simulink model "A3_4_vrx"  (R2024b)
settings: Solver=ode4  StartTime=0.0  StopTime=T_run  FixedStep=Ts_ctrl  RelTol=1e-3
InitFcn:
  | if ~exist('A3_model_init','file'), addpath(fileparts(get_param('A3_4_vrx','FileName'))); end, A3_model_init('A3_4_vrx')
StopFcn:
  | A3_model_done('A3_4_vrx')
values from neighbouring files (symbols this model uses):
  alloc_mode = 2    [A3_setup.m]
  animate = 0    [A3_setup.m]
  az_prm = [half_beam; l_thr; F_max; d_max; rev_on]    [A3_setup.m]
  d_rate = deg2rad(d_rate_deg)    [A3_setup.m]
  F_max = 500    [A3_azpolar_example.m]    (also in A3_nullspace_example.m; A3_pinv_example.m; A3_setup.m)
  Kb = Ki_u/Kp_u    (= 0.333333333333)    [A3_setup.m]
  Kd_psi = 200    [A3_setup.m]
  Ki_u = 100    [A3_setup.m]
  Ki_v = 100    [A3_setup.m]
  Kp_psi = 400    [A3_setup.m]
  Kp_u = 300    [A3_setup.m]
  Kp_v = 300    [A3_setup.m]
  Kp_x = 0.4    [A3_setup.m]
  Kp_y = 0.4    [A3_setup.m]
  N_max = 2*half_beam*F_max    (= 1027.135)    [A3_setup.m]
  origin_east = 0    [A3_setup.m]
  origin_north = 0    [A3_setup.m]
  R_stop = 1.5    [A3_setup.m]
  stop_hold = 15    [A3_setup.m]
  stop_q = [x_d; y_d; psi_d]    [A3_setup.m]
  svo_rate = deg2rad(svo_rate_deg)    [A3_setup.m]
  svo_tau = svo_tau_s    (= 0.2)    [A3_setup.m]
  Ts_ctrl = 0.05    [A3_setup.m]
  u_max = 1.5    [A3_setup.m]
  U_stop = 0.05    [A3_setup.m]
  v_max = 0.6    [A3_setup.m]
  vrx_pos_sign = -1    [A3_setup.m]
  Y_max = F_max / T_per_Y    [A3_setup.m]
libraries: ros2lib x9, slpidlib x2
settings Model: Creator=admin  LastModifiedBy=admin

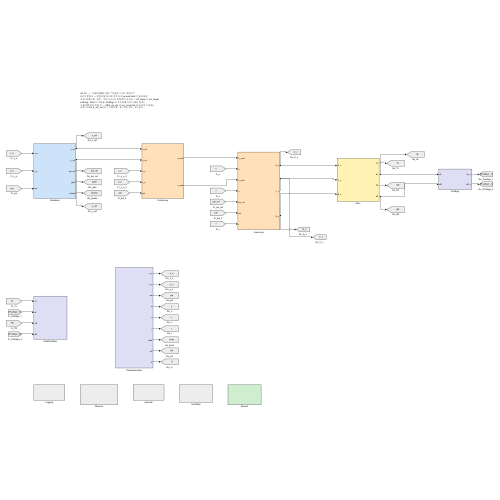
[thumbnail: Simulink's stored preview of the top-level diagram]
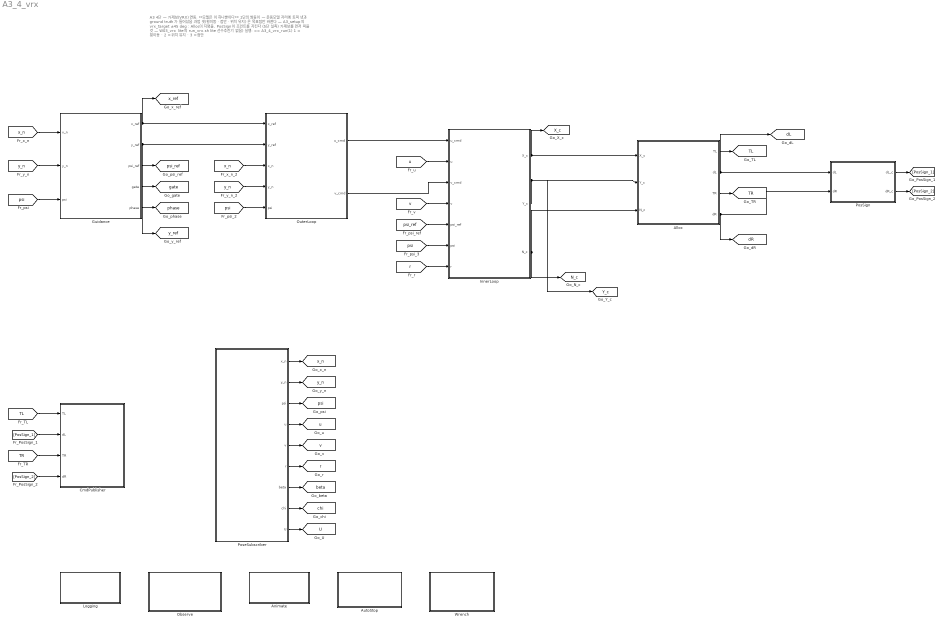
== system A3_4_vrx ==
  note: A3 4단  —  가제보(VRX) 연동. **모델은 이 하나뿐이다**
      | 2단의 쌍둥이 — 운동모델 자리에 토픽 넷과 ground truth 가 들어섰음
      | 과업 셋(횡이동 · 접안 · 위치 유지) 은 목표점만 바뀐다 — A3_setup 의 vrx_target
      | ±45 deg : Alloc 이 지령을, PosSign 이 조인트를 지킨다 (5단 실측)
      | 가제보를 먼저 띄울 것 — W03_vrx_lite 의 run_vrx.sh lite (선수추진기 없음)
      | 실행: >> A3_4_vrx_run(1)   1 = 횡이동 · 2 = 위치 유지 · 3 = 접안
  Alloc : Subsystem
  Animate : Subsystem
  AutoStop : Subsystem
  CmdPublisher : Subsystem
  Guidance : Subsystem
  InnerLoop : Subsystem
  Logging : Subsystem
  Observe : Subsystem
  OuterLoop : Subsystem
  PosSign : Subsystem
  PoseSubscriber : Subsystem
  Wrench : Subsystem
  tag scope: N_c=global, TL=global, TR=global, U=global, X_c=global, Y_c=global, beta=global, chi=global, dL=global, dR=global, gate=global, phase=global, psi=global, psi_ref=global, r=global, u=global, v=global, x_n=global, x_ref=global, y_n=global, y_ref=global
  wires:
  InnerLoop/2(Y_c) -> [Y_c], Alloc/2(Y_c)
  OuterLoop/1(u_cmd) -> InnerLoop/1(u_cmd)
  Alloc/2(dL) -> PosSign/1(dL), [dL]
  InnerLoop/1(X_c) -> Alloc/1(X_c), [X_c]
  OuterLoop/2(v_cmd) -> InnerLoop/3(v_cmd)
  Guidance/2(y_ref) -> OuterLoop/2(y_ref), [y_ref]
  Guidance/1(x_ref) -> OuterLoop/1(x_ref), [x_ref]
  PosSign/1(dL_c) -> [PosSign_1]
  PosSign/2(dR_c) -> [PosSign_2]
  Alloc/1(TL) -> [TL]
  Alloc/3(TR) -> [TR]
  PoseSubscriber/3(psi) -> [psi]
  Guidance/3(psi_ref) -> [psi_ref]
  PoseSubscriber/6(r) -> [r]
  PoseSubscriber/4(u) -> [u]
  PoseSubscriber/5(v) -> [v]
  PoseSubscriber/1(x_n) -> [x_n]
  PoseSubscriber/2(y_n) -> [y_n]
  [PosSign_1] -> CmdPublisher/2(dL)
  [PosSign_2] -> CmdPublisher/4(dR)
  [TL] -> CmdPublisher/1(TL)
  [TR] -> CmdPublisher/3(TR)
  [psi] -> Guidance/3(psi)
  [r] -> InnerLoop/7(r)
  [u] -> InnerLoop/2(u)
  [x_n] -> Guidance/1(x_n)
  [x_n] -> OuterLoop/3(x_n)
  [y_n] -> Guidance/2(y_n)
  [y_n] -> OuterLoop/4(y_n)
  PoseSubscriber/9(U) -> [U]
  PoseSubscriber/7(beta) -> [beta]
  PoseSubscriber/8(chi) -> [chi]
  Guidance/4(gate) -> [gate]
  Guidance/5(phase) -> [phase]
  [psi] -> OuterLoop/5(psi)
  [psi] -> InnerLoop/6(psi)
  [psi_ref] -> InnerLoop/5(psi_ref)
  [v] -> InnerLoop/4(v)
  Alloc/4(dR) -> [dR], PosSign/2(dR)
  InnerLoop/3(N_c) -> Alloc/3(N_c), [N_c]

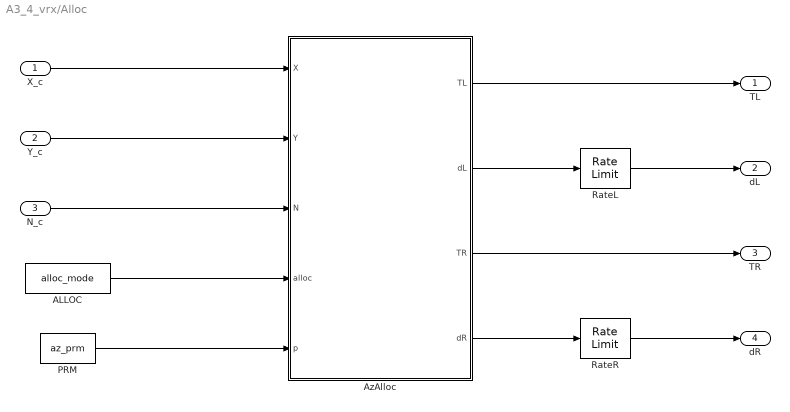
== system A3_4_vrx/Alloc ==
  X_c : Inport
  Y_c : Inport  Port=2
  N_c : Inport  Port=3
  ALLOC : Constant  Value=alloc_mode
  AzAlloc : MATLAB Function  TreatAsAtomicUnit=on
  PRM : Constant  Value=az_prm
  RateL : RateLimiter  RisingSlewLimit=d_rate  FallingSlewLimit=-d_rate  SampleTimeMode=inherited
  RateR : RateLimiter  RisingSlewLimit=d_rate  FallingSlewLimit=-d_rate  SampleTimeMode=inherited
  TL : Outport
  dL : Outport  Port=2
  TR : Outport  Port=3
  dR : Outport  Port=4
  wires:
  X_c/1 -> AzAlloc/1(X)
  Y_c/1 -> AzAlloc/2(Y)
  N_c/1 -> AzAlloc/3(N)
  ALLOC/1 -> AzAlloc/4(alloc)
  PRM/1 -> AzAlloc/5(p)
  AzAlloc/2(dL) -> RateL/1
  AzAlloc/4(dR) -> RateR/1
  AzAlloc/1(TL) -> TL/1
  RateL/1 -> dL/1
  RateR/1 -> dR/1
  AzAlloc/3(TR) -> TR/1

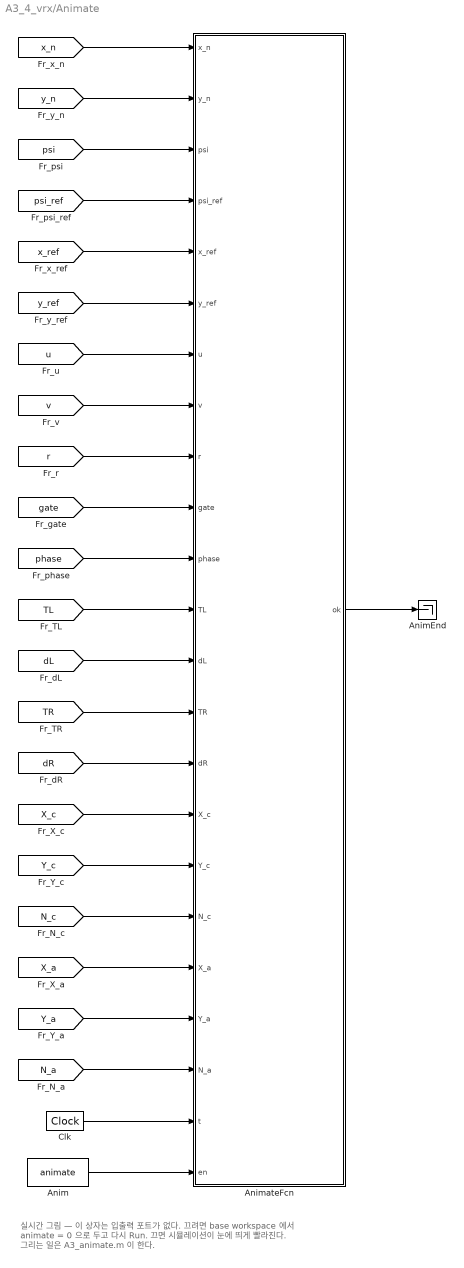
== system A3_4_vrx/Animate ==
  note: 실시간 그림 — 이 상자는 입출력 포트가 없다.
      | 끄려면 base workspace 에서  animate = 0  으로 두고 다시 Run.
      | 끄면 시뮬레이션이 눈에 띄게 빨라진다.
      | 그리는 일은 A3_animate.m 이 한다.
  Anim : Constant  Value=animate
  AnimEnd : Terminator
  AnimateFcn : MATLAB Function  TreatAsAtomicUnit=on
  Clk : DigitalClock  SampleTime=Ts_ctrl
  wires:
  [x_n] -> AnimateFcn/1(x_n)
  [y_n] -> AnimateFcn/2(y_n)
  [psi] -> AnimateFcn/3(psi)
  [psi_ref] -> AnimateFcn/4(psi_ref)
  [x_ref] -> AnimateFcn/5(x_ref)
  [y_ref] -> AnimateFcn/6(y_ref)
  [u] -> AnimateFcn/7(u)
  [v] -> AnimateFcn/8(v)
  [r] -> AnimateFcn/9(r)
  [gate] -> AnimateFcn/10(gate)
  [phase] -> AnimateFcn/11(phase)
  [TL] -> AnimateFcn/12(TL)
  [dL] -> AnimateFcn/13(dL)
  [TR] -> AnimateFcn/14(TR)
  [dR] -> AnimateFcn/15(dR)
  [X_c] -> AnimateFcn/16(X_c)
  [Y_c] -> AnimateFcn/17(Y_c)
  [N_c] -> AnimateFcn/18(N_c)
  [X_a] -> AnimateFcn/19(X_a)
  [Y_a] -> AnimateFcn/20(Y_a)
  [N_a] -> AnimateFcn/21(N_a)
  Clk/1 -> AnimateFcn/22(t)
  Anim/1 -> AnimateFcn/23(en)
  AnimateFcn/1(ok) -> AnimEnd/1

== system A3_4_vrx/AutoStop ==
  Done : RelationalOperator  OutDataTypeStr=boolean  RndMeth=Simplest  InputSameDT=off
  HeldFor : Integrator  ExternalReset=level
  Hold : Constant  Value=stop_hold
  One : Constant
  StopSim : Stop
  wires:
  One/1 -> HeldFor/1
  [gate] -> HeldFor/2
  HeldFor/1 -> Done/1
  Hold/1 -> Done/2
  Done/1 -> StopSim/1

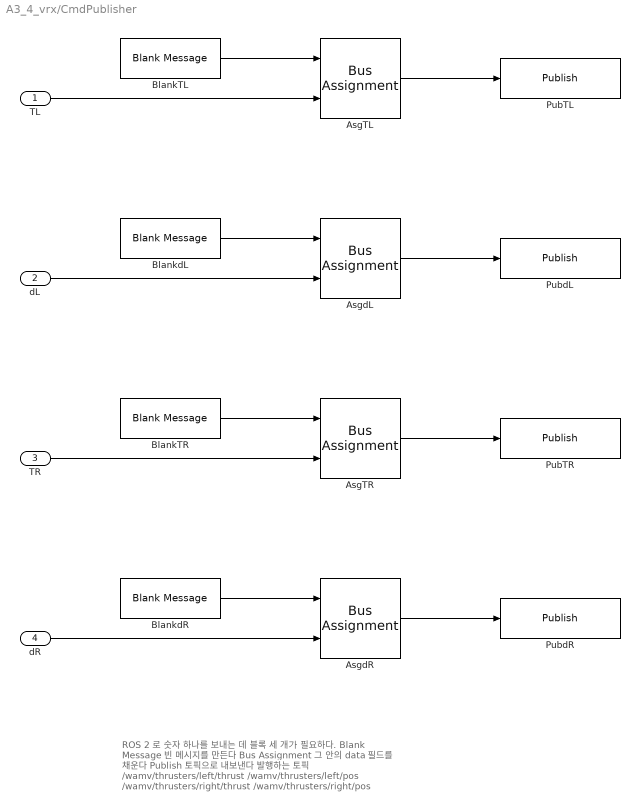
== system A3_4_vrx/CmdPublisher ==
  note: ROS 2 로 숫자 하나를 보내는 데 블록 세 개가 필요하다.
      |   Blank Message   빈 메시지를 만든다
      |   Bus Assignment  그 안의 data 필드를 채운다
      |   Publish         토픽으로 내보낸다
      |
      | 발행하는 토픽
      | /wamv/thrusters/left/thrust
      | /wamv/thrusters/left/pos
      | /wamv/thrusters/right/thrust
      | /wamv/thrusters/right/pos
  TL : Inport
  dL : Inport  Port=2
  TR : Inport  Port=3
  dR : Inport  Port=4
  AsgTL : BusAssignment  AssignedSignals=data
  AsgTR : BusAssignment  AssignedSignals=data
  AsgdL : BusAssignment  AssignedSignals=data
  AsgdR : BusAssignment  AssignedSignals=data
  BlankTL : ros2lib/Blank Message  messageClass=Message  entityType=std_msgs/Float64  messageType=std_msgs/Float64  SampleTime=Ts_ctrl
  BlankTR : ros2lib/Blank Message  messageClass=Message  entityType=std_msgs/Float64  messageType=std_msgs/Float64  SampleTime=Ts_ctrl
  BlankdL : ros2lib/Blank Message  messageClass=Message  entityType=std_msgs/Float64  messageType=std_msgs/Float64  SampleTime=Ts_ctrl
  BlankdR : ros2lib/Blank Message  messageClass=Message  entityType=std_msgs/Float64  messageType=std_msgs/Float64  SampleTime=Ts_ctrl
  PubTL : ros2lib/Publish  topicSource=Specify your own  topic=/wamv/thrusters/left/thrust  messageType=std_msgs/Float64  QOSHistory=Keep last  QOSDepth=1  QOSReliability=Reliable  QOSDurability=Volatile  QOSDeadline=Inf  QOSLifespan=Inf  QOSLiveliness=Automatic  QOSLeaseDuration=Inf  QOSAvoidROSNamespaceConventions=off
  PubTR : ros2lib/Publish  topicSource=Specify your own  topic=/wamv/thrusters/right/thrust  messageType=std_msgs/Float64  QOSHistory=Keep last  QOSDepth=1  QOSReliability=Reliable  QOSDurability=Volatile  QOSDeadline=Inf  QOSLifespan=Inf  QOSLiveliness=Automatic  QOSLeaseDuration=Inf  QOSAvoidROSNamespaceConventions=off
  PubdL : ros2lib/Publish  topicSource=Specify your own  topic=/wamv/thrusters/left/pos  messageType=std_msgs/Float64  QOSHistory=Keep last  QOSDepth=1  QOSReliability=Reliable  QOSDurability=Volatile  QOSDeadline=Inf  QOSLifespan=Inf  QOSLiveliness=Automatic  QOSLeaseDuration=Inf  QOSAvoidROSNamespaceConventions=off
  PubdR : ros2lib/Publish  topicSource=Specify your own  topic=/wamv/thrusters/right/pos  messageType=std_msgs/Float64  QOSHistory=Keep last  QOSDepth=1  QOSReliability=Reliable  QOSDurability=Volatile  QOSDeadline=Inf  QOSLifespan=Inf  QOSLiveliness=Automatic  QOSLeaseDuration=Inf  QOSAvoidROSNamespaceConventions=off
  wires:
  BlankTL/1 -> AsgTL/1
  AsgTL/1 -> PubTL/1
  TL/1 -> AsgTL/2
  BlankdL/1 -> AsgdL/1
  AsgdL/1 -> PubdL/1
  dL/1 -> AsgdL/2
  BlankTR/1 -> AsgTR/1
  AsgTR/1 -> PubTR/1
  TR/1 -> AsgTR/2
  BlankdR/1 -> AsgdR/1
  AsgdR/1 -> PubdR/1
  dR/1 -> AsgdR/2

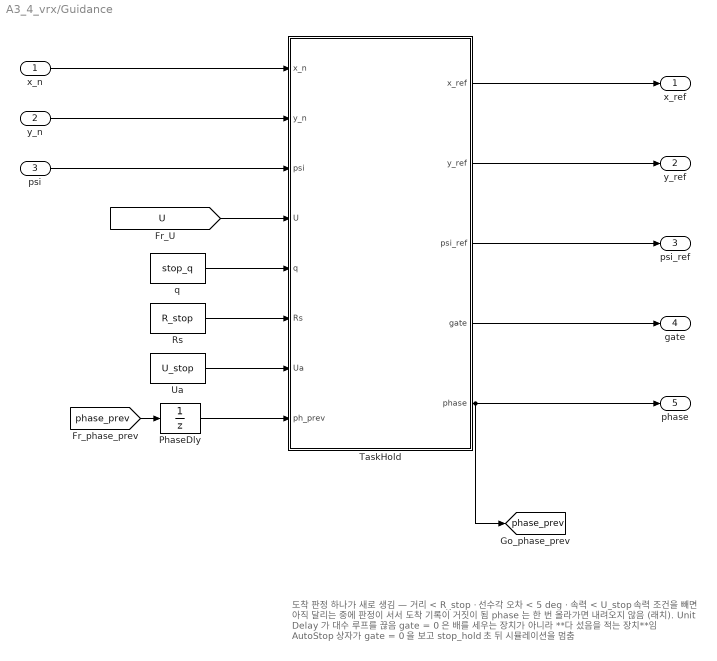
== system A3_4_vrx/Guidance ==
  note: 도착 판정 하나가 새로 생김 — 거리 < R_stop · 선수각 오차 < 5 deg · 속력 < U_stop
      | 속력 조건을 빼면 아직 달리는 중에 판정이 서서 도착 기록이 거짓이 됨
      | phase 는 한 번 올라가면 내려오지 않음 (래치). Unit Delay 가 대수 루프를 끊음
      | gate = 0 은 배를 세우는 장치가 아니라 **다 섰음을 적는 장치**임
      | AutoStop 상자가 gate = 0 을 보고 stop_hold 초 뒤 시뮬레이션을 멈춤
  x_n : Inport
  y_n : Inport  Port=2
  psi : Inport  Port=3
  PhaseDly : UnitDelay  Description=phase 래치가 자기 자신을 입력으로 받으므로 그대로 되먹이면 대수 루프가 된다. 한 스텝 전 값을 쓰는 것 말고는 끊을 방법이 없는 자리다. 표본 간격을 고정 스텝(Ts_ctrl)과 같게 두어 연속 솔버(ode4)와 어긋나지 않는다.  SampleTime=Ts_ctrl  HasFrameUpgradeWarning=on
  Rs : Constant  Value=R_stop
  TaskHold : MATLAB Function  TreatAsAtomicUnit=on
  Ua : Constant  Value=U_stop
  q : Constant  Value=stop_q
  x_ref : Outport
  y_ref : Outport  Port=2
  psi_ref : Outport  Port=3
  gate : Outport  Port=4
  phase : Outport  Port=5
  tag scope: phase_prev=global
  wires:
  x_n/1 -> TaskHold/1(x_n)
  y_n/1 -> TaskHold/2(y_n)
  psi/1 -> TaskHold/3(psi)
  [U] -> TaskHold/4(U)
  q/1 -> TaskHold/5(q)
  Rs/1 -> TaskHold/6(Rs)
  Ua/1 -> TaskHold/7(Ua)
  PhaseDly/1 -> TaskHold/8(ph_prev)
  TaskHold/1(x_ref) -> x_ref/1
  TaskHold/2(y_ref) -> y_ref/1
  TaskHold/3(psi_ref) -> psi_ref/1
  TaskHold/4(gate) -> gate/1
  TaskHold/5(phase) -> phase/1, [phase_prev]
  [phase_prev] -> PhaseDly/1

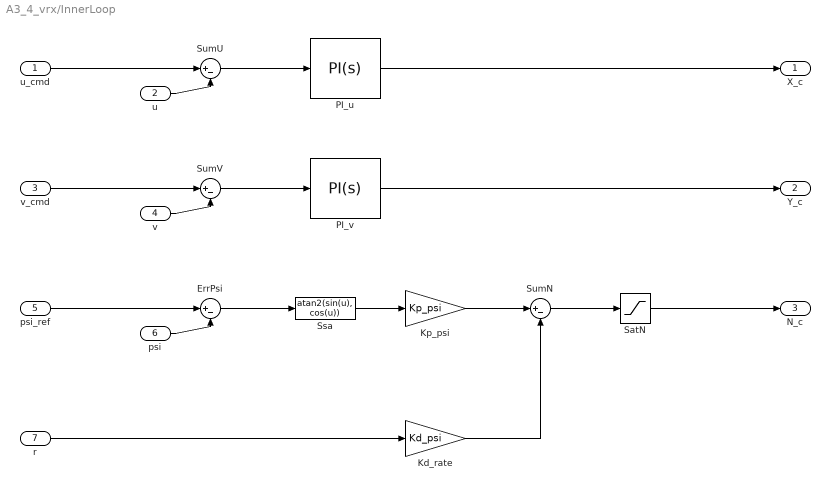
== system A3_4_vrx/InnerLoop ==
  u_cmd : Inport
  u : Inport  Port=2
  v_cmd : Inport  Port=3
  v : Inport  Port=4
  psi_ref : Inport  Port=5
  psi : Inport  Port=6
  r : Inport  Port=7
  ErrPsi : Sum  Inputs=|+-
  Kd_rate : Gain  Gain=Kd_psi
  Kp_psi : Gain  Gain=Kp_psi
  PI_u : slpidlib/PID Controller  Controller=PI  Form=Parallel  TimeDomain=Continuous-time  UseExternalTs=off  SampleTime=-1  IntegratorMethod=Forward Euler  FilterMethod=Forward Euler  ControllerParametersSource=internal  P=Kp_u  I=Ki_u  UseKiTs=off  D=0  UseExternalDerivativeSource=off  N=100  UseFilter=on  TunerSelectOption=Transfer Function Based (PID Tuner App)  InitialConditionSource=internal  InitialConditionForIntegrator=0  InitialConditionForFilter=0  DifferentiatorICPrevScaledInput=0  ExternalReset=none  TrackingMode=off  Kt=1  LimitOutput=on  SatLimitsSource=internal  UpperSaturationLimit=2*F_max  LowerSaturationLimit=-(2*F_max)  LinearizeAsGain=on  AntiWindupMode=back-calculation  Kb=Kb  LimitIntegrator=off  UpperIntegratorSaturationLimit=inf  LowerIntegratorSaturationLimit=-inf  POutMin=[]  POutMax=[]  IOutMin=[]  IOutMax=[]  DOutMin=[]  DOutMax=[]  NOutMin=[]  NOutMax=[]  SumOutMin=[]  SumOutMax=[]  SaturationOutMin=[]  SaturationOutMax=[]  PParamMin=[]  PParamMax=[]  IParamMin=[]  IParamMax=[]  DParamMin=[]  DParamMax=[]  NParamMin=[]  NParamMax=[]  KbParamMin=[]  KbParamMax=[]  KtParamMin=[]  KtParamMax=[]  KbOutMin=[]  KbOutMax=[]  KtOutMin=[]  KtOutMax=[]  IntegratorOutMin=[]  IntegratorOutMax=[]  FilterOutMin=[]  FilterOutMax=[]  SumI1OutMin=[]  SumI1OutMax=[]  SumI2OutMin=[]  SumI2OutMax=[]  SumI3OutMin=[]  SumI3OutMax=[]  SumI4OutMin=[]  SumI4OutMax=[]  SumDOutMin=[]  SumDOutMax=[]  DifferentiatorOutMin=[]  DifferentiatorOutMax=[]  FilterDiffOutCoefMin=[]  FilterDiffOutCoefMax=[]  ReciprocalOutMin=[]  ReciprocalOutMax=[]  SumDenOutMin=[]  SumDenOutMax=[]  SumNumOutMin=[]  SumNumOutMax=[]  DivideOutMin=[]  DivideOutMax=[]  UdiffTsProdOutMin=[]  UdiffTsProdOutMax=[]  NTsProdOutMin=[]  NTsProdOutMax=[]  UintegralTsProdOutMin=[]  UintegralTsProdOutMax=[]  UngainTsProdOutMin=[]  UngainTsProdOutMax=[]  ClampingZeroOutDataTypeStr=Inherit: Inherit via back propagation  ClampingZeroOutMin=[]  ClampingZeroOutMax=[]  FilterDenConstantOutDataTypeStr=Inherit: Inherit via back propagation  FilterDenConstantOutMin=[]  FilterDenConstantOutMax=[]  PCopyOutDataTypeStr=Inherit: Inherit via back propagation  PCopyOutMin=[]  PCopyOutMax=[]  NCopyOutDataTypeStr=Inherit: Inherit via back propagation  NCopyOutMin=[]  NCopyOutMax=[]  IntegratorContinuousStateAttributes=''  IntegratorStateMustResolveToSignalObject=off  IntegratorRTWStateStorageClass=Auto  FilterContinuousStateAttributes=''  FilterStateMustResolveToSignalObject=off  FilterRTWStateStorageClass=Auto  ParallelPVariant=InternalParameters  IdealPVariant=Disabled  IVariant=InternalParameters  DVariant=Disabled  IntegratorVariant=Continuous  SatVariant=Enabled  AWVariant=BackCalculation  PCopyVariant=Disabled  TRVariant=Disabled  FdbkBlocksVariant=Forward  IdealPFdbkVariant=Disabled  SatFdbkVariant=Disabled  DerivativeFilterVariant=Disabled  NVariant=Disabled  NCopyVariant=Disabled_SignalSpec  FilterICVariant=Disabled  IntegratorICVariant=InternalICs  ExternalResetVariant=Disabled  TRSumVariant=Passthrough  SumFdbkVariant=Disabled  SumVariant=Sum_PI  TsampFilterVariant=InternalTs  TsampNgainVariant=Passthrough  TsampIntegralVariant=Disabled_SignalSpec  ExternalSaturationOutDataTypeStr=Inherit: Same as second input  DerivativeSourceVariant=Disabled  PreIntVariant=InternalPreInt
  PI_v : slpidlib/PID Controller  Controller=PI  Form=Parallel  TimeDomain=Continuous-time  UseExternalTs=off  SampleTime=-1  IntegratorMethod=Forward Euler  FilterMethod=Forward Euler  ControllerParametersSource=internal  P=Kp_v  I=Ki_v  UseKiTs=off  D=0  UseExternalDerivativeSource=off  N=100  UseFilter=on  TunerSelectOption=Transfer Function Based (PID Tuner App)  InitialConditionSource=internal  InitialConditionForIntegrator=0  InitialConditionForFilter=0  DifferentiatorICPrevScaledInput=0  ExternalReset=none  TrackingMode=off  Kt=1  LimitOutput=on  SatLimitsSource=internal  UpperSaturationLimit=Y_max  LowerSaturationLimit=-(Y_max)  LinearizeAsGain=on  AntiWindupMode=back-calculation  Kb=Kb  LimitIntegrator=off  UpperIntegratorSaturationLimit=inf  LowerIntegratorSaturationLimit=-inf  POutMin=[]  POutMax=[]  IOutMin=[]  IOutMax=[]  DOutMin=[]  DOutMax=[]  NOutMin=[]  NOutMax=[]  SumOutMin=[]  SumOutMax=[]  SaturationOutMin=[]  SaturationOutMax=[]  PParamMin=[]  PParamMax=[]  IParamMin=[]  IParamMax=[]  DParamMin=[]  DParamMax=[]  NParamMin=[]  NParamMax=[]  KbParamMin=[]  KbParamMax=[]  KtParamMin=[]  KtParamMax=[]  KbOutMin=[]  KbOutMax=[]  KtOutMin=[]  KtOutMax=[]  IntegratorOutMin=[]  IntegratorOutMax=[]  FilterOutMin=[]  FilterOutMax=[]  SumI1OutMin=[]  SumI1OutMax=[]  SumI2OutMin=[]  SumI2OutMax=[]  SumI3OutMin=[]  SumI3OutMax=[]  SumI4OutMin=[]  SumI4OutMax=[]  SumDOutMin=[]  SumDOutMax=[]  DifferentiatorOutMin=[]  DifferentiatorOutMax=[]  FilterDiffOutCoefMin=[]  FilterDiffOutCoefMax=[]  ReciprocalOutMin=[]  ReciprocalOutMax=[]  SumDenOutMin=[]  SumDenOutMax=[]  SumNumOutMin=[]  SumNumOutMax=[]  DivideOutMin=[]  DivideOutMax=[]  UdiffTsProdOutMin=[]  UdiffTsProdOutMax=[]  NTsProdOutMin=[]  NTsProdOutMax=[]  UintegralTsProdOutMin=[]  UintegralTsProdOutMax=[]  UngainTsProdOutMin=[]  UngainTsProdOutMax=[]  ClampingZeroOutDataTypeStr=Inherit: Inherit via back propagation  ClampingZeroOutMin=[]  ClampingZeroOutMax=[]  FilterDenConstantOutDataTypeStr=Inherit: Inherit via back propagation  FilterDenConstantOutMin=[]  FilterDenConstantOutMax=[]  PCopyOutDataTypeStr=Inherit: Inherit via back propagation  PCopyOutMin=[]  PCopyOutMax=[]  NCopyOutDataTypeStr=Inherit: Inherit via back propagation  NCopyOutMin=[]  NCopyOutMax=[]  IntegratorContinuousStateAttributes=''  IntegratorStateMustResolveToSignalObject=off  IntegratorRTWStateStorageClass=Auto  FilterContinuousStateAttributes=''  FilterStateMustResolveToSignalObject=off  FilterRTWStateStorageClass=Auto  ParallelPVariant=InternalParameters  IdealPVariant=Disabled  IVariant=InternalParameters  DVariant=Disabled  IntegratorVariant=Continuous  SatVariant=Enabled  AWVariant=BackCalculation  PCopyVariant=Disabled  TRVariant=Disabled  FdbkBlocksVariant=Forward  IdealPFdbkVariant=Disabled  SatFdbkVariant=Disabled  DerivativeFilterVariant=Disabled  NVariant=Disabled  NCopyVariant=Disabled_SignalSpec  FilterICVariant=Disabled  IntegratorICVariant=InternalICs  ExternalResetVariant=Disabled  TRSumVariant=Passthrough  SumFdbkVariant=Disabled  SumVariant=Sum_PI  TsampFilterVariant=InternalTs  TsampNgainVariant=Passthrough  TsampIntegralVariant=Disabled_SignalSpec  ExternalSaturationOutDataTypeStr=Inherit: Same as second input  DerivativeSourceVariant=Disabled  PreIntVariant=InternalPreInt
  SatN : Saturate  UpperLimit=N_max  LowerLimit=-(N_max)
  Ssa : Fcn  Expr=atan2(sin(u), cos(u))
  SumN : Sum  Inputs=|+-
  SumU : Sum  Inputs=|+-
  SumV : Sum  Inputs=|+-
  X_c : Outport
  Y_c : Outport  Port=2
  N_c : Outport  Port=3
  wires:
  u_cmd/1 -> SumU/1
  u/1 -> SumU/2
  v_cmd/1 -> SumV/1
  v/1 -> SumV/2
  SumU/1 -> PI_u/1
  SumV/1 -> PI_v/1
  ErrPsi/1 -> Ssa/1
  psi_ref/1 -> ErrPsi/1
  psi/1 -> ErrPsi/2
  Ssa/1 -> Kp_psi/1
  r/1 -> Kd_rate/1
  Kp_psi/1 -> SumN/1
  Kd_rate/1 -> SumN/2
  SumN/1 -> SatN/1
  PI_u/1 -> X_c/1
  SatN/1 -> N_c/1
  PI_v/1 -> Y_c/1

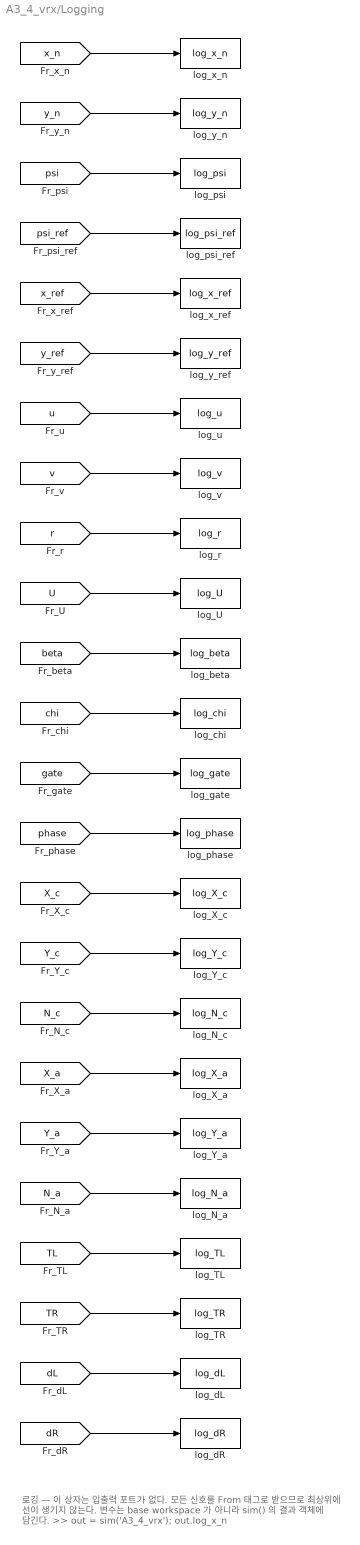
== system A3_4_vrx/Logging ==
  note: 로깅 — 이 상자는 입출력 포트가 없다.
      | 모든 신호를 From 태그로 받으므로 최상위에 선이 생기지 않는다.
      | 변수는 base workspace 가 아니라 sim() 의 결과 객체에 담긴다.
      |   >> out = sim('A3_4_vrx');  out.log_x_n
  log_N_a : ToWorkspace  VariableName=log_N_a  SaveFormat=Timeseries  SampleTime=Ts_ctrl
  log_N_c : ToWorkspace  VariableName=log_N_c  SaveFormat=Timeseries  SampleTime=Ts_ctrl
  log_TL : ToWorkspace  VariableName=log_TL  SaveFormat=Timeseries  SampleTime=Ts_ctrl
  log_TR : ToWorkspace  VariableName=log_TR  SaveFormat=Timeseries  SampleTime=Ts_ctrl
  log_U : ToWorkspace  VariableName=log_U  SaveFormat=Timeseries  SampleTime=Ts_ctrl
  log_X_a : ToWorkspace  VariableName=log_X_a  SaveFormat=Timeseries  SampleTime=Ts_ctrl
  log_X_c : ToWorkspace  VariableName=log_X_c  SaveFormat=Timeseries  SampleTime=Ts_ctrl
  log_Y_a : ToWorkspace  VariableName=log_Y_a  SaveFormat=Timeseries  SampleTime=Ts_ctrl
  log_Y_c : ToWorkspace  VariableName=log_Y_c  SaveFormat=Timeseries  SampleTime=Ts_ctrl
  log_beta : ToWorkspace  VariableName=log_beta  SaveFormat=Timeseries  SampleTime=Ts_ctrl
  log_chi : ToWorkspace  VariableName=log_chi  SaveFormat=Timeseries  SampleTime=Ts_ctrl
  log_dL : ToWorkspace  VariableName=log_dL  SaveFormat=Timeseries  SampleTime=Ts_ctrl
  log_dR : ToWorkspace  VariableName=log_dR  SaveFormat=Timeseries  SampleTime=Ts_ctrl
  log_gate : ToWorkspace  VariableName=log_gate  SaveFormat=Timeseries  SampleTime=Ts_ctrl
  log_phase : ToWorkspace  VariableName=log_phase  SaveFormat=Timeseries  SampleTime=Ts_ctrl
  log_psi : ToWorkspace  VariableName=log_psi  SaveFormat=Timeseries  SampleTime=Ts_ctrl
  log_psi_ref : ToWorkspace  VariableName=log_psi_ref  SaveFormat=Timeseries  SampleTime=Ts_ctrl
  log_r : ToWorkspace  VariableName=log_r  SaveFormat=Timeseries  SampleTime=Ts_ctrl
  log_u : ToWorkspace  VariableName=log_u  SaveFormat=Timeseries  SampleTime=Ts_ctrl
  log_v : ToWorkspace  VariableName=log_v  SaveFormat=Timeseries  SampleTime=Ts_ctrl
  log_x_n : ToWorkspace  VariableName=log_x_n  SaveFormat=Timeseries  SampleTime=Ts_ctrl
  log_x_ref : ToWorkspace  VariableName=log_x_ref  SaveFormat=Timeseries  SampleTime=Ts_ctrl
  log_y_n : ToWorkspace  VariableName=log_y_n  SaveFormat=Timeseries  SampleTime=Ts_ctrl
  log_y_ref : ToWorkspace  VariableName=log_y_ref  SaveFormat=Timeseries  SampleTime=Ts_ctrl
  wires:
  [x_n] -> log_x_n/1
  [y_n] -> log_y_n/1
  [psi] -> log_psi/1
  [psi_ref] -> log_psi_ref/1
  [x_ref] -> log_x_ref/1
  [y_ref] -> log_y_ref/1
  [u] -> log_u/1
  [v] -> log_v/1
  [r] -> log_r/1
  [U] -> log_U/1
  [beta] -> log_beta/1
  [chi] -> log_chi/1
  [gate] -> log_gate/1
  [phase] -> log_phase/1
  [X_c] -> log_X_c/1
  [Y_c] -> log_Y_c/1
  [N_c] -> log_N_c/1
  [X_a] -> log_X_a/1
  [Y_a] -> log_Y_a/1
  [N_a] -> log_N_a/1
  [TL] -> log_TL/1
  [TR] -> log_TR/1
  [dL] -> log_dL/1
  [dR] -> log_dR/1

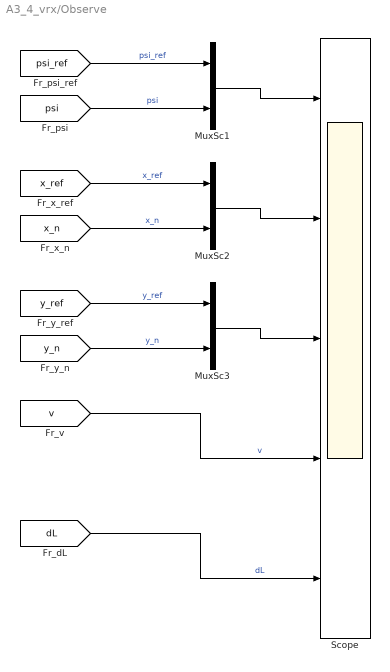
== system A3_4_vrx/Observe ==
  MuxSc1 : Mux  Inputs=2
  MuxSc2 : Mux  Inputs=2
  MuxSc3 : Mux  Inputs=2
  Scope : Scope  NumInputPorts=5
  wires:
  [psi_ref] -> MuxSc1/1  "psi_ref"
  [psi] -> MuxSc1/2  "psi"
  MuxSc1/1 -> Scope/1
  [x_ref] -> MuxSc2/1  "x_ref"
  [x_n] -> MuxSc2/2  "x_n"
  MuxSc2/1 -> Scope/2
  [y_ref] -> MuxSc3/1  "y_ref"
  [y_n] -> MuxSc3/2  "y_n"
  MuxSc3/1 -> Scope/3
  [v] -> Scope/4  "v"
  [dL] -> Scope/5  "dL"

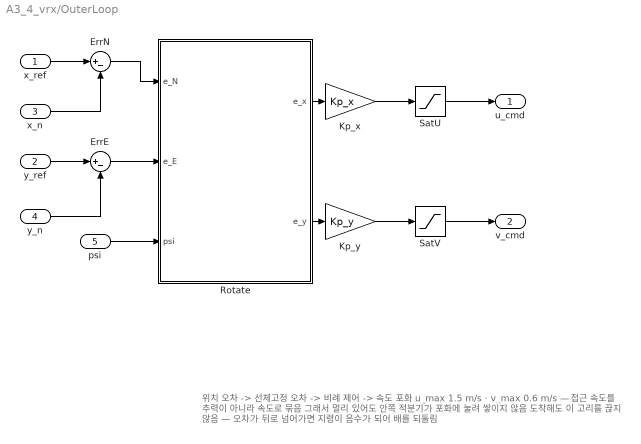
== system A3_4_vrx/OuterLoop ==
  note: 위치 오차 -> 선체고정 오차 -> 비례 제어 -> 속도 포화
      | u_max 1.5 m/s · v_max 0.6 m/s — 접근 속도를 추력이 아니라 속도로 묶음
      | 그래서 멀리 있어도 안쪽 적분기가 포화에 눌려 쌓이지 않음
      | 도착해도 이 고리를 끊지 않음 — 오차가 뒤로 넘어가면 지령이 음수가 되어 배를 되돌림
  x_ref : Inport
  y_ref : Inport  Port=2
  x_n : Inport  Port=3
  y_n : Inport  Port=4
  psi : Inport  Port=5
  ErrE : Sum  Inputs=|+-
  ErrN : Sum  Inputs=|+-
  Kp_x : Gain  Gain=Kp_x
  Kp_y : Gain  Gain=Kp_y
  Rotate : MATLAB Function  TreatAsAtomicUnit=on
  SatU : Saturate  UpperLimit=u_max  LowerLimit=-(u_max)
  SatV : Saturate  UpperLimit=v_max  LowerLimit=-(v_max)
  u_cmd : Outport
  v_cmd : Outport  Port=2
  wires:
  x_ref/1 -> ErrN/1
  x_n/1 -> ErrN/2
  ErrE/1 -> Rotate/2(e_E)
  y_ref/1 -> ErrE/1
  y_n/1 -> ErrE/2
  Rotate/1(e_x) -> Kp_x/1
  ErrN/1 -> Rotate/1(e_N)
  psi/1 -> Rotate/3(psi)
  Rotate/2(e_y) -> Kp_y/1
  Kp_x/1 -> SatU/1
  Kp_y/1 -> SatV/1
  SatU/1 -> u_cmd/1
  SatV/1 -> v_cmd/1

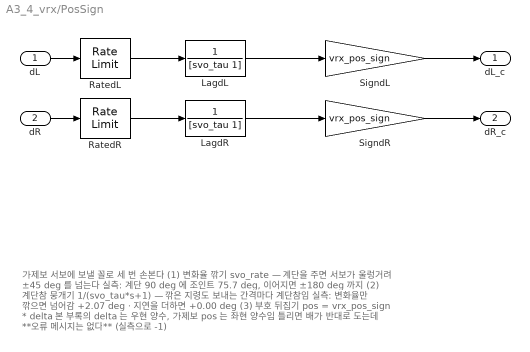
== system A3_4_vrx/PosSign ==
  note: 가제보 서보에 보낼 꼴로 세 번 손본다
      | (1) 변화율 깎기 svo_rate — 계단을 주면 서보가 울렁거려 ±45 deg 를 넘는다
      |       실측: 계단 90 deg 에 조인트 75.7 deg, 이어지면 ±180 deg 까지
      | (2) 계단참 뭉개기 1/(svo_tau*s+1) — 깎은 지령도 보내는 간격마다 계단참임
      |       실측: 변화율만 깎으면 넘어감 +2.07 deg · 지연을 더하면 +0.00 deg
      | (3) 부호 뒤집기 pos = vrx_pos_sign * delta
      |       본 부록의 delta 는 우현 양수, 가제보 pos 는 좌현 양수임
      |       틀리면 배가 반대로 도는데 **오류 메시지는 없다** (실측으로 -1)
  dL : Inport
  dR : Inport  Port=2
  LagdL : TransferFcn  Denominator=[svo_tau 1]
  LagdR : TransferFcn  Denominator=[svo_tau 1]
  RatedL : RateLimiter  RisingSlewLimit=svo_rate  FallingSlewLimit=-svo_rate  SampleTimeMode=inherited
  RatedR : RateLimiter  RisingSlewLimit=svo_rate  FallingSlewLimit=-svo_rate  SampleTimeMode=inherited
  SigndL : Gain  Gain=vrx_pos_sign
  SigndR : Gain  Gain=vrx_pos_sign
  dL_c : Outport
  dR_c : Outport  Port=2
  wires:
  dL/1 -> RatedL/1
  RatedL/1 -> LagdL/1
  LagdL/1 -> SigndL/1
  SigndL/1 -> dL_c/1
  dR/1 -> RatedR/1
  RatedR/1 -> LagdR/1
  LagdR/1 -> SigndR/1
  SigndR/1 -> dR_c/1

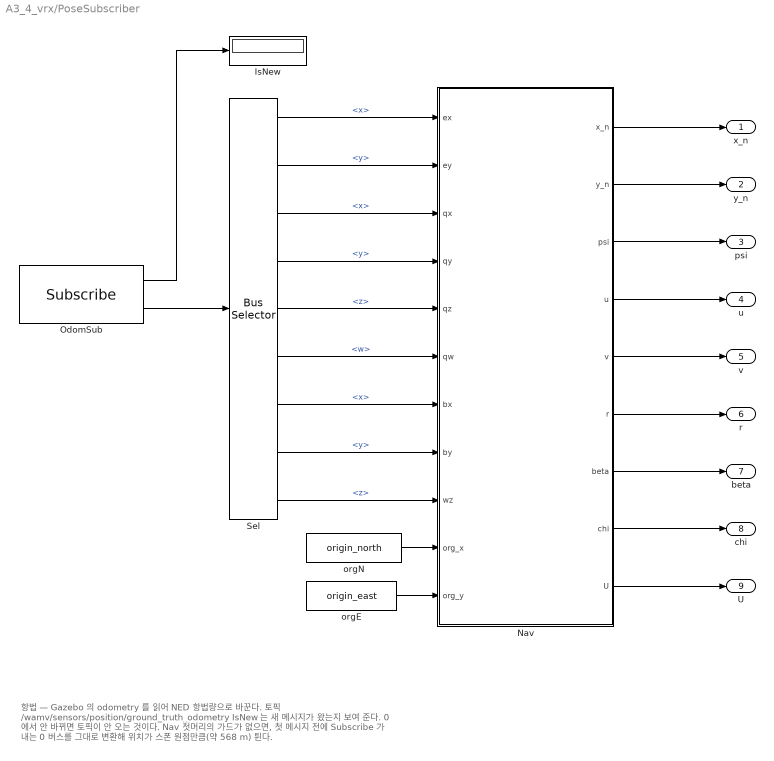
== system A3_4_vrx/PoseSubscriber ==
  note: 항법 — Gazebo 의 odometry 를 읽어 NED 항법량으로 바꾼다.
      |   토픽 /wamv/sensors/position/ground_truth_odometry
      |
      | IsNew 는 새 메시지가 왔는지 보여 준다. 0 에서 안 바뀌면 토픽이 안 오는 것이다.
      | Nav 첫머리의 가드가 없으면, 첫 메시지 전에 Subscribe 가 내는 0 버스를
      | 그대로 변환해 위치가 스폰 원점만큼(약 568 m) 튄다.
  IsNew : Display
  Nav : MATLAB Function  TreatAsAtomicUnit=on
  OdomSub : ros2lib/Subscribe  topicSource=Specify your own  topic=/wamv/sensors/position/ground_truth_odometry  messageType=nav_msgs/Odometry  sampleTime=Ts_ctrl  QOSHistory=Keep last  QOSDepth=1  QOSReliability=Reliable  QOSDurability=Volatile  QOSDeadline=Inf  QOSLifespan=Inf  QOSLiveliness=Automatic  QOSLeaseDuration=Inf  QOSAvoidROSNamespaceConventions=off
  Sel : BusSelector  OutputSignals=pose.pose.position.x,pose.pose.position.y,pose.pose.orientation.x,pose.pose.orientation.y,pose.pose.orientation.z,pose.pose.orientation.w,twist.twist.linear.x,twist.twist.linear.y,twist.twist.angular.z
  orgE : Constant  Value=origin_east
  orgN : Constant  Value=origin_north
  x_n : Outport
  y_n : Outport  Port=2
  psi : Outport  Port=3
  u : Outport  Port=4
  v : Outport  Port=5
  r : Outport  Port=6
  beta : Outport  Port=7
  chi : Outport  Port=8
  U : Outport  Port=9
  wires:
  OdomSub/1 -> IsNew/1
  OdomSub/2 -> Sel/1
  Sel/1 -> Nav/1(ex)  "<x>"
  Sel/2 -> Nav/2(ey)  "<y>"
  Sel/3 -> Nav/3(qx)  "<x>"
  Sel/4 -> Nav/4(qy)  "<y>"
  Sel/5 -> Nav/5(qz)  "<z>"
  Sel/6 -> Nav/6(qw)  "<w>"
  Sel/7 -> Nav/7(bx)  "<x>"
  Sel/8 -> Nav/8(by)  "<y>"
  Sel/9 -> Nav/9(wz)  "<z>"
  orgN/1 -> Nav/10(org_x)
  orgE/1 -> Nav/11(org_y)
  Nav/1(x_n) -> x_n/1
  Nav/2(y_n) -> y_n/1
  Nav/3(psi) -> psi/1
  Nav/4(u) -> u/1
  Nav/5(v) -> v/1
  Nav/6(r) -> r/1
  Nav/7(beta) -> beta/1
  Nav/8(chi) -> chi/1
  Nav/9(U) -> U/1

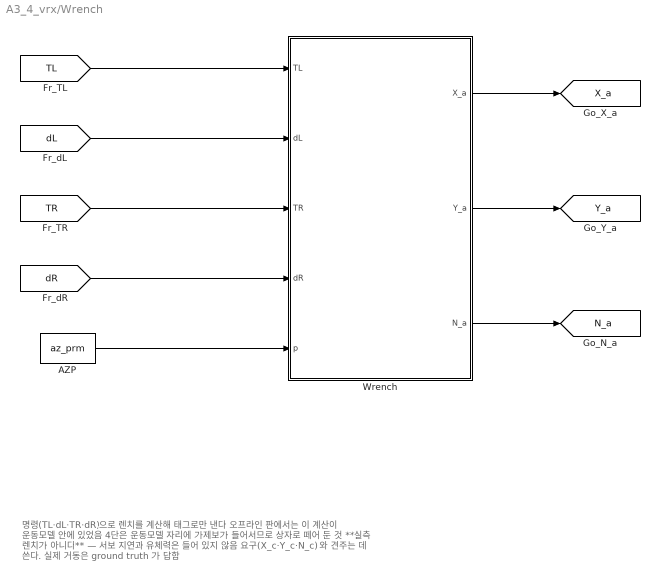
== system A3_4_vrx/Wrench ==
  note: 명령(TL·dL·TR·dR)으로 렌치를 계산해 태그로만 낸다
      | 오프라인 판에서는 이 계산이 운동모델 안에 있었음
      | 4단은 운동모델 자리에 가제보가 들어서므로 상자로 떼어 둔 것
      | **실측 렌치가 아니다** — 서보 지연과 유체력은 들어 있지 않음
      | 요구(X_c·Y_c·N_c) 와 견주는 데 쓴다. 실제 거동은 ground truth 가 답함
  AZP : Constant  Value=az_prm
  Wrench : MATLAB Function  TreatAsAtomicUnit=on
  tag scope: N_a=global, X_a=global, Y_a=global
  wires:
  [TL] -> Wrench/1(TL)
  [dL] -> Wrench/2(dL)
  [TR] -> Wrench/3(TR)
  [dR] -> Wrench/4(dR)
  AZP/1 -> Wrench/5(p)
  Wrench/1(X_a) -> [X_a]
  Wrench/2(Y_a) -> [Y_a]
  Wrench/3(N_a) -> [N_a]

== matlab function A3_4_vrx/Animate/AnimateFcn ==
  data: x_n input; y_n input; psi input; psi_ref input; x_ref input; y_ref input; u input; ok output; v input; r input; gate input; phase input; TL input; dL input; TR input; dR input; X_c input; Y_c input; N_c input; X_a input; Y_a input; N_a input; t input; en input
function ok = AnimateFcn(x_n, y_n, psi, psi_ref, x_ref, y_ref, u, v, r, gate, phase, TL, dL, TR, dR, X_c, Y_c, N_c, X_a, Y_a, N_a, t, en)
%#codegen
% Live plot while the model runs. A MATLAB Function block cannot
% plot, so the drawing function is declared extrinsic: Simulink
% calls plain MATLAB instead of generating code for it.
coder.extrinsic('A3_animate');
ok = 1;
if en > 0.5
    A3_animate(x_n, y_n, psi, psi_ref, x_ref, y_ref, u, v, r, gate, phase, TL, dL, TR, dR, X_c, Y_c, N_c, X_a, Y_a, N_a, t);
end

== matlab function A3_4_vrx/OuterLoop/Rotate ==
  data: e_N input; e_x output; e_E input; psi input; e_y output
function [e_x, e_y] = Rotate(e_N, e_E, psi)
%#codegen
%  NED 위치 오차를 선체고정 오차로 돌린다. e_x 앞쪽, e_y 우현쪽 [m]
e_x =  cos(psi)*e_N + sin(psi)*e_E;
e_y = -sin(psi)*e_N + cos(psi)*e_E;

== matlab function A3_4_vrx/Guidance/TaskHold ==
  data: x_n input; x_ref output; y_n input; psi input; U input; q input; Rs input; Ua input; ph_prev input; y_ref output; psi_ref output; gate output; phase output
function [x_ref, y_ref, psi_ref, gate, phase] = TaskHold(x_n, y_n, psi, U, q, Rs, Ua, ph_prev)
%#codegen
%  한 점·한 선수각을 목표로 주고, 거기 가서 **섰는지** 판정한다.
%
%    U  = 대지속력 [m/s]      운동모델이 낸 sqrt(u^2 + v^2)
%    q  = [x_d; y_d; psi_d]   목표 자세 (psi_d 는 rad)
%    Rs = R_stop              도착으로 보는 반지름 [m]
%    Ua = U_stop              도착으로 보는 속력 한계 [m/s]
%
%  gate = 1 이면 바깥 고리가 속도 지령을 낸다. 0 이면 0 을 내어 배가 선다.
x_ref = q(1);  y_ref = q(2);  psi_ref = q(3);
d = sqrt((x_ref - x_n)^2 + (y_ref - y_n)^2);
e = atan2(sin(psi_ref - psi), cos(psi_ref - psi));
ph = ph_prev;
if ph < 1 && d < Rs && abs(e) < 5*pi/180 && U < Ua
    ph = 1;                   %  도착 — 한 번 올라가면 내려오지 않는다
end
phase = ph;
gate  = double(ph < 1);

== matlab function A3_4_vrx/Alloc/AzAlloc ==
  data: X input; TL output; Y input; N input; alloc input; p input; dL output; TR output; dR output
function [TL, dL, TR, dR] = AzAlloc(X, Y, N, alloc, p)
%#codegen
%  아지무스 추진기 둘에 요구 렌치를 나누어 준다
%
%  == 입력 ==============================================================
%    X      요구 전후 힘   [N]      선수 방향(+앞)
%    Y      요구 횡 힘     [N]      우현 방향(+오른쪽)
%    N      요구 요 모멘트 [N m]    시계 방향(+우선회)
%    alloc  배분 방식 [-]           1 = pseudo-inverse
%                                   2 = pseudo-inverse + null space 보정
%    p      기하·한계 묶음 (A3_setup.m 의 az_prm)
%      p(1) = b     반폭        [m]    중심선에서 추진기까지
%      p(2) = L     거리        [m]    무게중심에서 추진기까지 (뒤쪽)
%      p(3) = Fmax  추력 한계   [N]    한 대 기준
%      p(4) = dmax  각도 한계   [rad]
%      p(5) = rev   추력 반전   [-]    1 = 허용, 0 = 금지
%
%  == 출력 ==============================================================
%    TL, TR   좌·우 추력   [N]    양수면 노즐이 보는 쪽으로 민다
%    dL, dR   좌·우 각도   [rad]  선수 기준, 우현 쪽이 +
%
%  == 왜 추력과 각도를 바로 풀지 않는가 ================================
%    추진기 한 대의 힘은 극좌표 (T, d) 로 쓰면 비선형이다
%        Fx = T cos(d),   Fy = T sin(d)
%    그래서 추력과 각도를 묶어 **직교 성분 넷**을 미지수로 둔다
%        ue = [Fx_L; Fy_L; Fx_R; Fy_R]        (확장 추력 벡터)
%    이렇게 두면 요구 렌치와의 관계가 **완전한 선형식**이 된다
%        B ue = tau,   tau = [X; Y; N]
%    B 의 각 열은 "그 성분 1 N 이 렌치에 얼마를 보태는가" 이다
%    풀고 난 뒤에 극좌표로 되돌리면 추력과 각도가 나온다 (3 단계)
%    이 방식은 Sarda 등 [1] 6 절이 실제 WAM-V 에 쓴 것과 같다
%
%  == 해가 하나가 아니다 ================================================
%    미지수 4 개, 식 3 개 — 같은 렌치를 내는 해가 **직선 하나**를 이룬다
%      alloc = 1   그 직선에서 원점에 가장 가까운 점 (pseudo-inverse)
%      alloc = 2   각도 한계를 지키는 점으로 직선 위를 미끄러진다
%    직선의 방향 n = [0; 1; 0; -1] 은 좌우 횡력만 주고받는 꼴이라
%    얼마를 더해도 X, Y, N 이 한 톨도 변하지 않는다 (B n = 0)
%
%  == 참고 문헌 ==========================================================
%    [1] Sarda, Qu, Bertaska, von Ellenrieder (2016)
%        "Station keeping control of an unmanned surface vehicle exposed
%         to current and wind disturbances", Ocean Engineering 127, 305-324
%        6 절 — 아지무스 WAM-V 의 확장 추력 벡터와 pseudo-inverse 배분
%    [2] Sordalen (1997) "Optimal thrust allocation for marine vessels",
%        Control Engineering Practice 5(9), 1223-1231 — null space 이용
%    [3] Fossen (2021) "Handbook of Marine Craft Hydrodynamics and Motion
%        Control", 2nd ed., 11 장 — 배분 행렬과 pseudo-inverse 일반론

b = p(1);  L = p(2);  Fmax = p(3);  dmax = p(4);  rev = p(5);

tau = [X; Y; N];

%  배분 행렬 — 열 하나가 성분 하나의 몫이다
%    1 행 전후 · 2 행 횡 · 3 행 요 모멘트
%    좌현은 (x, y) = (-L, -b), 우현은 (-L, +b) 에 앉는다
B = [ 1,  0,  1,  0; ...
      0,  1,  0,  1; ...
      b, -L, -b, -L];

%  === 1 단계. pseudo-inverse — 크기가 가장 작은 해 ===================
%    ue = B' (B B')^-1 tau.  해의 직선에서 원점에 가장 가까운 점이다
ue = B' * ((B*B') \ tau);

%  === 2 단계. null space 보정 (alloc = 2) ============================
%    각도 한계는 |Fy| <= tan(dmax) |Fx| 와 같은 말이다.
%    ue + lam*n 을 넣으면 lam 에 대해 1 차식이라 허용 구간이 바로 나온다
if alloc > 1.5
    nz = [0; 1; 0; -1];
    td = tan(dmax);
    lo = max(-td*abs(ue(1)) - ue(2),  ue(4) - td*abs(ue(3)));
    hi = min( td*abs(ue(1)) - ue(2),  ue(4) + td*abs(ue(3)));
    if lo <= hi
        lam = min(max(0, lo), hi);     % 구간 안에서 0 에 가장 가까운 값
    else
        lam = (lo + hi)/2;             % 구간이 비면 가운데 — 덜 넘긴다
    end
    ue = ue + lam*nz;
end

%  === 3 단계. 극좌표로 되돌리고 한계 안으로 넣는다 ===================
[TL, dL] = az_polar(ue(1), ue(2), Fmax, dmax, rev);
[TR, dR] = az_polar(ue(3), ue(4), Fmax, dmax, rev);


function [T, d] = az_polar(Fx, Fy, Fmax, dmax, rev)
%  직교 성분 둘 -> 추력 하나와 각도 하나
T = hypot(Fx, Fy);
d = atan2(Fy, Fx);

%  뒤쪽을 보라는 요구는 **앞을 보고 역추력** 으로 바꿔 쓴다 (같은 힘)
if abs(d) > pi/2
    d = d - sign(d)*pi;
    T = -T;
end

%  역추력을 금지했으면 되돌린다 — 각도가 한계를 넘게 된다 (A3-4 실습)
if rev < 0.5 && T < 0
    T = -T;
    d = d + sign(d + (d==0))*pi;
    if d >  pi, d = d - 2*pi; end
    if d < -pi, d = d + 2*pi; end
end

%  한계 — 각도와 추력을 각각 한 줄로 깎는다
%    깎인 만큼이 "못 낸 힘" 으로 남아 운동모델 쪽 기록에 숫자로 보인다
d = max(min(d,  dmax), -dmax);
T = max(min(T,  Fmax), -Fmax);

== matlab function A3_4_vrx/PoseSubscriber/Nav ==
  data: ex input; x_n output; ey input; qx input; qy input; qz input; qw input; bx input; by input; wz input; org_x input; org_y input; y_n output; psi output; u output; v output; r output; beta output; chi output; U output
function [x_n, y_n, psi, u, v, r, beta, chi, U] = Nav(ex, ey, qx, qy, qz, qw, bx, by, wz, org_x, org_y)
%#codegen
%  Gazebo/ROS 는 ENU 에 선체축 x 앞 · y 좌현 · z 위.
%  해양제어는 NED 에 선체축 x 앞 · y 우현 · z 아래.
%
%    위치   : 북 = y_ENU,  동 = x_ENU   (스폰 원점을 뺀다)
%    선수각 : psi = pi/2 - yaw_ENU
%    선체속도: u = bx,  v = -by,  r = -wz   (y·z 부호가 바뀐다)

%  첫 메시지가 오기 전 Subscribe 는 0 으로 채운 버스를 낸다. 그대로 쓰면
%  위치가 스폰 원점만큼(수백 m) 튀어 로그 첫 점이 망가진다.
if ex == 0 && ey == 0
    x_n = 0; y_n = 0; psi = 0; u = 0; v = 0; r = 0; beta = 0; chi = 0; U = 0;
    return
end
x_n = ey - org_x;    % north, 스폰 기준 상대좌표
y_n = ex - org_y;    % east

yaw_enu = atan2(2*(qw*qz + qx*qy), 1 - 2*(qy*qy + qz*qz));
p   = pi/2 - yaw_enu;
psi = atan2(sin(p), cos(p));

u = bx;
v = -by;
r = -wz;

U    = sqrt(u*u + v*v);
beta = atan2(v, u);          % 크랩각
c    = psi + beta;
chi  = atan2(sin(c), cos(c));

== matlab function A3_4_vrx/Wrench/Wrench ==
  data: TL input; X_a output; dL input; TR input; dR input; p input; Y_a output; N_a output
function [X_a, Y_a, N_a] = Wrench(TL, dL, TR, dR, p)
%#codegen
%  추진기 명령 -> 선체에 걸리는 렌치 (운동모델의 입구)
%
%  == 입력 ==============================================================
%    TL, TR   좌·우 추력 [N]      배분기가 낸 값. 음수면 역추력
%    dL, dR   좌·우 각도 [rad]    변화율 제한을 거친 실제 각도
%    p        기하 묶음 — p(1) = b 반폭 [m], p(2) = L 거리 [m]
%
%  == 출력 ==============================================================
%    X_a  실제 전후 힘   [N]
%    Y_a  실제 횡 힘     [N]
%    N_a  실제 요 모멘트 [N m]
%
%  == 왜 운동모델 안에 있는가 ===========================================
%    선체가 받는 것은 추력과 각도가 아니라 **힘과 모멘트**다. 추진기가
%    어떻게 달려 있는지가 그 변환을 정하므로, 변환은 배(운동모델) 쪽에
%    속한다. 배분기는 "무엇을 명령할까" 까지만 책임진다
%
%  == 배분기와 같은 행렬이다 ============================================
%    배분기는 B ue = tau 를 **거꾸로** 풀었고, 여기서는 **바로** 쓴다
%        ue = [TL cos(dL); TL sin(dL); TR cos(dR); TR sin(dR)]
%        tau_a = B ue
%    각도·추력 한계에 물리지 않으면 tau_a 가 요구 렌치와 같아진다.
%    기하를 고칠 때는 azAllocFcn.m 의 B 와 **함께** 고쳐야 한다

b = p(1);  L = p(2);

B = [ 1,  0,  1,  0; ...
      0,  1,  0,  1; ...
      b, -L, -b, -L];

%  극좌표(추력·각도) -> 직교 성분 넷
ue = [TL*cos(dL); TL*sin(dL); TR*cos(dR); TR*sin(dR)];

tau_a = B*ue;

X_a = tau_a(1);  Y_a = tau_a(2);  N_a = tau_a(3);
